simulink model "SZ03_ERR"  (R2026a)
settings: Solver=VariableStepAuto  MaxStep=tau/25
InitFcn:
  | K = 5;
  | tau = 0.125;
  | 
  | y_0 = -0.5;
settings Model: Creator=Szalay  LastModifiedBy=Szalay

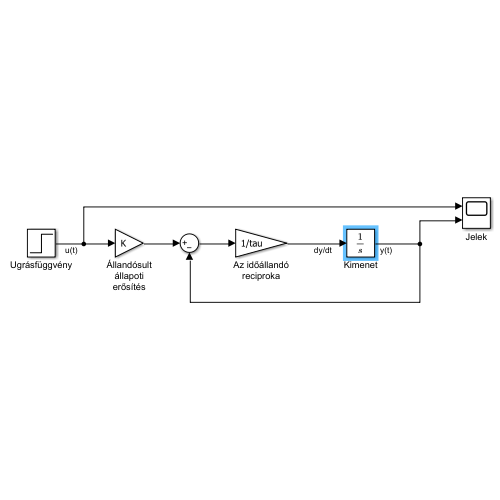
[thumbnail: Simulink's stored preview of the top-level diagram]
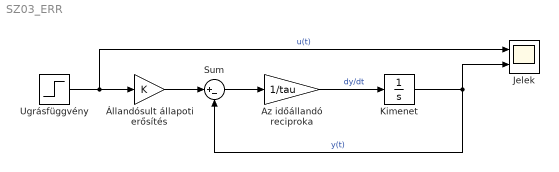
== system SZ03_ERR ==
  Az időállandó reciproka : Gain  Gain=1/tau
  Jelek : Scope  NumInputPorts=2
      settings: ActiveDisplayYMinimum=-1.183285943021819  ActiveDisplayYMaximum=5.6495734871963723
  Kimenet : Integrator  InitialCondition=y_0
  Sum : Sum  Inputs=|+-
  Ugrásfüggvény : Step  Time=5  SampleTime=0
  Állandósult állapoti erősítés : Gain  Gain=K
  wires:
  Kimenet/1 -> Sum/2, Jelek/2  "y(t)"
  Az időállandó reciproka/1 -> Kimenet/1  "dy/dt"
  Sum/1 -> Az időállandó reciproka/1
  Állandósult állapoti erősítés/1 -> Sum/1
  Ugrásfüggvény/1 -> Jelek/1, Állandósult állapoti erősítés/1  "u(t)"
